simulink model "Mission_Server_Swarm_2QDrone"  (Simulink 9.1)
settings: Solver=ode2  StartTime=0.0  StopTime=inf  FixedStep=0.001  RelTol=1e-3  EnableMultiTasking=on
undefined symbols (not defined in the file): Host, qc_get_step_size
libraries: quarc_library x31, simulink x8
(part 2 of 2)

== system Mission_Server_Swarm_2QDrone/MISSION SERVER QDRONE SWARM/Communications Check/Triggered Subsystem1 ==
  note: This looks for the first falling edge to trigger a communication issue,
      | because the mission server model starts first.
  Trigger : TriggerPort  TriggerType=falling  VariantControl=Variant
  Add : Sum
  Compare To Constant : simulink/Logic and Bit Operations/Compare To Constant  relop=>=  const=1  OutDataTypeStr=boolean
  Constant : Constant
  Memory : Memory  InheritSampleTime=on
  Communication Issue (0,1) : Outport  InitialOutput=0
  wires:
  Compare To Constant/1 -> Communication Issue (0,1)/1
  Add/1 -> Memory/1, Compare To Constant/1
  Memory/1 -> Add/2
  Constant/1 -> Add/1

== system Mission_Server_Swarm_2QDrone/MISSION SERVER QDRONE SWARM/Data Server (Localization) /Convention Correction (Motive Frame to Research Studio Frame) - Drone 1 ==
  note: MF_R_RSF
  note: This subsystem converts measurements in the Motive Frame (MF)(raw optitrack) into the Research Studio Frame (RSF).
  note: RSF_R_MF
  note: XYZ in MF
  note: RPY in MF
  note: position
  note: attitude
  note: XYZ in RSF
  note: RPY in RSF
  xyz_MF (m) [3] : Inport
  rot_MF (rad) [3] : Inport  Port=2
  Inverse of  Orthonormal  Matrix is its  Transpose : Math  Operator=transpose  SaturateOnIntegerOverflow=on
  Prevent Gimbal Lock : Subsystem
  Product : Product  Multiplication=Matrix(*)
  Product1 : Product  Multiplication=Matrix(*)
  Rotate Basis from  RSF to MF : Constant  Value=[0 -1 0;0 0 1;-1 0 0]
  xyz_RSF (m) [3] : Outport
  rot_RSF (rad) [3] : Outport  Port=2
  wires:
  Rotate Basis from  RSF to MF/1 -> Inverse of  Orthonormal  Matrix is its  Transpose/1
  xyz_MF (m) [3]/1 -> Product1/2
  Inverse of  Orthonormal  Matrix is its  Transpose/1 -> Product1/1, Product/1
  rot_MF (rad) [3]/1 -> Product/2
  Product1/1 -> xyz_RSF (m) [3]/1
  Product/1 -> Prevent Gimbal Lock/1(Attitude (rad) [3])
  Prevent Gimbal Lock/1("Attitude (rad) [3] ") -> rot_RSF (rad) [3]/1

== system Mission_Server_Swarm_2QDrone/MISSION SERVER QDRONE SWARM/Data Server (Localization) /Convention Correction (Motive Frame to Research Studio Frame) - Drone 2 ==
  note: RPY in RSF
  note: XYZ in RSF
  note: attitude
  note: position
  note: RPY in MF
  note: XYZ in MF
  note: RSF_R_MF
  note: This subsystem converts measurements in the Motive Frame (MF)(raw optitrack) into the Research Studio Frame (RSF).
  note: MF_R_RSF
  xyz_MF (m) [3] : Inport
  rot_MF (rad) [3] : Inport  Port=2
  Inverse of  Orthonormal  Matrix is its  Transpose : Math  Operator=transpose  SaturateOnIntegerOverflow=on
  Prevent Gimbal Lock : Subsystem
  Product : Product  Multiplication=Matrix(*)
  Product1 : Product  Multiplication=Matrix(*)
  Rotate Basis from  RSF to MF : Constant  Value=[0 -1 0;0 0 1;-1 0 0]
  xyz_RSF (m) [3] : Outport
  rot_RSF (rad) [3] : Outport  Port=2
  wires:
  Prevent Gimbal Lock/1("Attitude (rad) [3] ") -> rot_RSF (rad) [3]/1
  Product/1 -> Prevent Gimbal Lock/1(Attitude (rad) [3])
  Product1/1 -> xyz_RSF (m) [3]/1
  rot_MF (rad) [3]/1 -> Product/2
  Inverse of  Orthonormal  Matrix is its  Transpose/1 -> Product/1, Product1/1
  xyz_MF (m) [3]/1 -> Product1/2
  Rotate Basis from  RSF to MF/1 -> Inverse of  Orthonormal  Matrix is its  Transpose/1

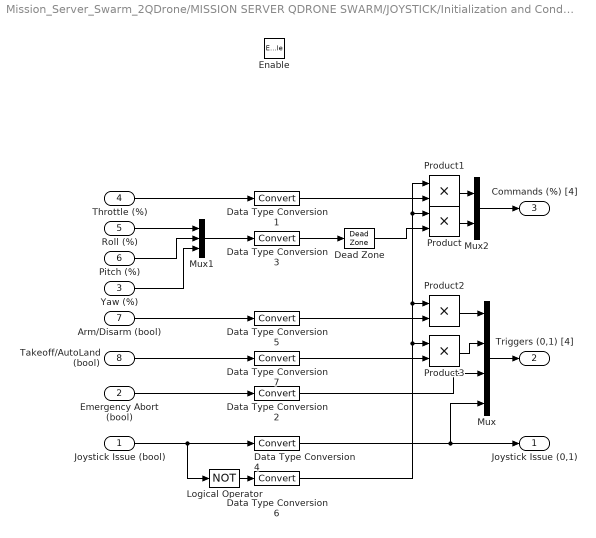
== system Mission_Server_Swarm_2QDrone/MISSION SERVER QDRONE SWARM/JOYSTICK/Initialization and Conditioning ==
  Joystick Issue (bool) : Inport
  Emergency Abort (bool) : Inport  Port=2
  Yaw (%) : Inport  Port=3
  Throttle (%) : Inport  Port=4
  Roll (%) : Inport  Port=5
  Pitch (%) : Inport  Port=6
  Arm/Disarm (bool) : Inport  Port=7
  Takeoff/AutoLand (bool) : Inport  Port=8
  Enable : EnablePort  StatesWhenEnabling=reset
  Data Type Conversion{1..7} (7 alike) : DataTypeConversion
  Dead Zone : DeadZone  LowerValue=-0.01  UpperValue=0.01  SaturateOnIntegerOverflow=on
  Logical Operator : Logic  Operator=NOT  AllPortsSameDT=off  OutDataTypeStr=boolean
  Mux : Mux
  Mux1 : Mux  Inputs=3
  Mux2 : Mux  Inputs=2
  Product{,1..3} (4 alike) : Product
  Joystick Issue (0,1) : Outport  InitialOutput=0
  Triggers (0,1) [4] : Outport  Port=2  InitialOutput=0
  Commands (%) [4] : Outport  Port=3  InitialOutput=0
  wires:
  Mux2/1 -> Commands (%) [4]/1
  Data Type Conversion7/1 -> Product3/2
  Product3/1 -> Mux/2
  Takeoff/AutoLand (bool)/1 -> Data Type Conversion7/1
  Data Type Conversion5/1 -> Product2/2
  Product2/1 -> Mux/1
  Data Type Conversion6/1 -> Product3/1, Product2/1, Product/1, Product1/1
  Dead Zone/1 -> Product/2
  Data Type Conversion1/1 -> Product1/2
  Product1/1 -> Mux2/1
  Product/1 -> Mux2/2
  Logical Operator/1 -> Data Type Conversion6/1
  Data Type Conversion2/1 -> Mux/3
  Mux/1 -> Triggers (0,1) [4]/1
  Arm/Disarm (bool)/1 -> Data Type Conversion5/1
  Data Type Conversion3/1 -> Dead Zone/1
  Emergency Abort (bool)/1 -> Data Type Conversion2/1
  Data Type Conversion4/1 -> Joystick Issue (0,1)/1, Mux/4
  Yaw (%)/1 -> Mux1/3
  Pitch (%)/1 -> Mux1/2
  Roll (%)/1 -> Mux1/1
  Throttle (%)/1 -> Data Type Conversion1/1
  Mux1/1 -> Data Type Conversion3/1
  Joystick Issue (bool)/1 -> Logical Operator/1, Data Type Conversion4/1

== system Mission_Server_Swarm_2QDrone/MISSION SERVER QDRONE SWARM/JOYSTICK/Pulse Check ==
  note: For this subsystem we will count the number of new pulses. The data can be considered enabled once the count of new signals has gone beyond 2. This will enable the Initializing and conditioning subsystem.
  new : Inport
  Compare : quarc_library/Logic Operations/Compare  operator=>  output_data_type=boolean
      settings: SourceProductName=QUARC Targets
  Pulse Check : Constant  Value=2
  "pulse count " : Subsystem  TreatAsAtomicUnit=on
  signal enable : Outport  InitialOutput=0
  wires:
  Compare/1 -> signal enable/1
  Pulse Check/1 -> Compare/2
  new/1 -> "pulse count "/Trigger
  "pulse count "/1(Number of Pulses) -> Compare/1

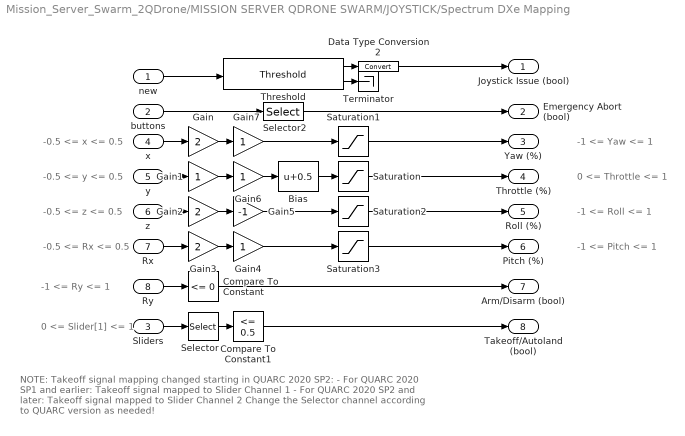
== system Mission_Server_Swarm_2QDrone/MISSION SERVER QDRONE SWARM/JOYSTICK/Spectrum DXe Mapping ==
  note: NOTE: Takeoff signal mapping changed starting in QUARC 2020 SP2:
      |
      | - For QUARC 2020 SP1 and earlier: Takeoff signal mapped to Slider Channel 1
      | - For QUARC 2020 SP2 and later: Takeoff signal mapped to Slider Channel 2
      |
      | Change the Selector channel according to QUARC version as needed!
  note: -1 <= Ry <= 1
  note: 0 <= Slider[1] <= 1
  note: -1 <= Pitch <= 1
  note: -0.5 <= Rx <= 0.5
  note: -1 <= Roll <= 1
  note: -0.5 <= z <= 0.5
  note: 0 <= Throttle <= 1
  note: -0.5 <= y <= 0.5
  note: -1 <= Yaw <= 1
  note: -0.5 <= x <= 0.5
  new : Inport
  buttons : Inport  Port=2
  Sliders : Inport  Port=3
  x : Inport  Port=4
  y : Inport  Port=5
  z : Inport  Port=6
  Rx : Inport  Port=7
  Ry : Inport  Port=8
  Bias : Bias  Bias=0.5
  Compare To Constant : simulink/Logic and Bit Operations/Compare To Constant  relop=<=  const=0  OutDataTypeStr=boolean
  Compare To Constant1 : simulink/Logic and Bit Operations/Compare To Constant  relop=<=  const=0.5  OutDataTypeStr=boolean
  Data Type Conversion2 : DataTypeConversion
  Gain : Gain  Gain=2
  Gain{1,4,6..7} (4 alike) : Gain
  Gain2 : Gain  Gain=2
  Gain3 : Gain  Gain=2
  Gain5 : Gain  Gain=-1
  Saturation : Saturate  UpperLimit=1  LowerLimit=0
  Saturation1 : Saturate  UpperLimit=1  LowerLimit=-1
  Saturation2 : Saturate  UpperLimit=1  LowerLimit=-1
  Saturation3 : Saturate  UpperLimit=1  LowerLimit=-1
  Selector : Selector  InputPortWidth=2  IndexOptions=Index vector (dialog)  Indices=[2]  OutputSizes=1
  Selector2 : Selector  InputPortWidth=32  IndexOptions=Index vector (dialog)  Indices=[1]  OutputSizes=1
  Terminator : Terminator
  Threshold : quarc_library/Discontinuities/Threshold  operator===  param_src=Specify via dialog  threshold=0  duration=1
      settings: SourceProductName=QUARC Targets
  Joystick Issue (bool) : Outport
  Emergency Abort (bool) : Outport  Port=2
  Yaw (%) : Outport  Port=3
  Throttle (%) : Outport  Port=4
  Roll (%) : Outport  Port=5
  Pitch (%) : Outport  Port=6
  "Arm/Disarm (bool) " : Outport  Port=7
  Takeoff/Autoland (bool) : Outport  Port=8
  wires:
  Data Type Conversion2/1 -> Joystick Issue (bool)/1
  new/1 -> Threshold/1
  Threshold/1 -> Data Type Conversion2/1
  Selector2/1 -> Emergency Abort (bool)/1
  Threshold/2 -> Terminator/1
  buttons/1 -> Selector2/1
  Compare To Constant1/1 -> Takeoff/Autoland (bool)/1
  Rx/1 -> Gain3/1
  y/1 -> Gain1/1
  Ry/1 -> Compare To Constant/1
  x/1 -> Gain/1
  z/1 -> Gain2/1
  Gain4/1 -> Saturation3/1
  Gain1/1 -> Gain6/1
  Gain2/1 -> Gain5/1
  Bias/1 -> Saturation/1
  Saturation2/1 -> Roll (%)/1
  Gain3/1 -> Gain4/1
  Gain/1 -> Gain7/1
  Saturation1/1 -> Yaw (%)/1
  Gain6/1 -> Bias/1
  Sliders/1 -> Selector/1
  Saturation/1 -> Throttle (%)/1
  Gain5/1 -> Saturation2/1
  Selector/1 -> Compare To Constant1/1
  Gain7/1 -> Saturation1/1
  Saturation3/1 -> Pitch (%)/1
  Compare To Constant/1 -> "Arm/Disarm (bool) "/1

== system Mission_Server_Swarm_2QDrone/MISSION SERVER QDRONE SWARM/Data Server (Localization) /Convention Correction (Motive Frame to Research Studio Frame) - Drone 1/Prevent Gimbal Lock ==
  note: Remapping the rotation order to prevent gimbal lock
      | in heading/yaw due to Euler singularity condition
  Attitude (rad) [3] : Inport
  Demux : Demux  Outputs=3
  Euler Angles from Rotation Matrix (Relative ZYX) : quarc_library/Math Operations/Matrices/Euler Angles from Rotation Matrix  menu_order=Relative Z-Y-X
      settings: SourceProductName=QUARC Targets
  Euler Angles to Rotation Matrix (Relative YZX) : quarc_library/Math Operations/Matrices/Euler Angles to Rotation Matrix  menu_order=Relative Y-Z-X
      settings: SourceProductName=QUARC Targets
  Mux : Mux  Inputs=3
  "Attitude (rad) [3] " : Outport
  wires:
  Euler Angles from Rotation Matrix (Relative ZYX)/2 -> Mux/2
  Euler Angles from Rotation Matrix (Relative ZYX)/1 -> Mux/3
  Euler Angles from Rotation Matrix (Relative ZYX)/3 -> Mux/1
  Euler Angles to Rotation Matrix (Relative YZX)/1 -> Euler Angles from Rotation Matrix (Relative ZYX)/1
  Attitude (rad) [3]/1 -> Demux/1
  Mux/1 -> "Attitude (rad) [3] "/1
  Demux/2 -> Euler Angles to Rotation Matrix (Relative YZX)/1
  Demux/3 -> Euler Angles to Rotation Matrix (Relative YZX)/2
  Demux/1 -> Euler Angles to Rotation Matrix (Relative YZX)/3

== system Mission_Server_Swarm_2QDrone/MISSION SERVER QDRONE SWARM/Data Server (Localization) /Convention Correction (Motive Frame to Research Studio Frame) - Drone 2/Prevent Gimbal Lock ==
  note: Remapping the rotation order to prevent gimbal lock
      | in heading/yaw due to Euler singularity condition
  Attitude (rad) [3] : Inport
  Demux : Demux  Outputs=3
  Euler Angles from Rotation Matrix (Relative ZYX) : quarc_library/Math Operations/Matrices/Euler Angles from Rotation Matrix  menu_order=Relative Z-Y-X
      settings: SourceProductName=QUARC Targets
  Euler Angles to Rotation Matrix (Relative YZX) : quarc_library/Math Operations/Matrices/Euler Angles to Rotation Matrix  menu_order=Relative Y-Z-X
      settings: SourceProductName=QUARC Targets
  Mux : Mux  Inputs=3
  "Attitude (rad) [3] " : Outport
  wires:
  Demux/1 -> Euler Angles to Rotation Matrix (Relative YZX)/3
  Demux/3 -> Euler Angles to Rotation Matrix (Relative YZX)/2
  Demux/2 -> Euler Angles to Rotation Matrix (Relative YZX)/1
  Mux/1 -> "Attitude (rad) [3] "/1
  Attitude (rad) [3]/1 -> Demux/1
  Euler Angles to Rotation Matrix (Relative YZX)/1 -> Euler Angles from Rotation Matrix (Relative ZYX)/1
  Euler Angles from Rotation Matrix (Relative ZYX)/3 -> Mux/1
  Euler Angles from Rotation Matrix (Relative ZYX)/1 -> Mux/3
  Euler Angles from Rotation Matrix (Relative ZYX)/2 -> Mux/2

== system Mission_Server_Swarm_2QDrone/MISSION SERVER QDRONE SWARM/JOYSTICK/Pulse Check/pulse count  ==
  Trigger : TriggerPort  VariantControl=Variant
  Constant1 : Constant  Value=0
  Increment Stored Integer : simulink/Additional Math & Discrete/Additional Math: Increment - Decrement/Increment Stored Integer
  Sum : Sum  Inputs=|++
  Unit Delay : UnitDelay  SampleTime=-1
  Number of Pulses : Outport
  wires:
  Constant1/1 -> Sum/1
  Sum/1 -> Increment Stored Integer/1
  Unit Delay/1 -> Sum/2
  Increment Stored Integer/1 -> Unit Delay/1, Number of Pulses/1

== matlab function MISSION SERVER QDRONE SWARM/n vehicles Circular Trajectories/generate vector of 0s for Yaw ==
  data: u input double; y output double
function y = fcn(u)

y = 0.*u;

== matlab function MISSION SERVER QDRONE SWARM/n vehicles Circular Trajectories/generate vector of 1s ==
  data: u input double; y output double
function y = fcn(u)

y = 0.*u + 1;

== matlab function MISSION SERVER QDRONE SWARM/n vehicles Circular Trajectories/variable size reshape ==
  data: u input double; y output double
function y = fcn(u)
y = u;
num = length(u)/4;
for i = 1:4
    for j = 1:num
        y(4*(j-1) + i) = u(j + num*(i-1));
    end
end

== matlab function Communication V1/Detect Communication loss/MATLAB Function ==
  data: time input double; stream_connection_loss output double; state input double; error input double
function stream_connection_loss  = fcn(time, state, error)

stream_connection_loss = 0;
if time > 1
    if ~((state == 2)&&(error >= 0))
        % stream connection is not established correctly
        stream_connection_loss = 1;
    end
end

== matlab function Communication V2/Detect Communication loss/MATLAB Function ==
  data: time input double; stream_connection_loss output double; state input double; error input double
function stream_connection_loss  = fcn(time, state, error)

stream_connection_loss = 0;
if time > 1
    if ~((state == 2)&&(error >= 0))
        % stream connection is not established correctly
        stream_connection_loss = 1;
    end
end

== matlab function MISSION SERVER QDRONE SWARM/Extract Vehicle Data 7/Extract Object Data ==
  data: data input double; position output double; orientation output double; index input double; tracking output double
function [position, orientation, tracking] = fcn(data, index)

n = length(data)/7;

if (index<=0)||(index>n)
    position = zeros(1,3); orientation = zeros(1,3); tracking = 0;
else
    position = [data(index*3-2), data(index*3-1), data(index*3)];
    orientation = [data((index+n)*3 - 2), data((index+n)*3 - 1), data((index+n)*3)];
    tracking = data(index + (n*6));
end

== matlab function MISSION SERVER QDRONE SWARM/Extract Vehicle Data 1/Extract Object Data ==
  data: data input double; position output double; orientation output double; index input double; tracking output double
function [position, orientation, tracking] = fcn(data, index)

n = length(data)/7;

if (index<=0)||(index>n)
    position = zeros(1,3); orientation = zeros(1,3); tracking = 0;
else
    position = [data(index*3-2), data(index*3-1), data(index*3)];
    orientation = [data((index+n)*3 - 2), data((index+n)*3 - 1), data((index+n)*3)];
    tracking = data(index + (n*6));
end

== matlab function MISSION SERVER QDRONE SWARM/Extract Vehicle Data 2/Extract Object Data ==
  data: data input double; position output double; orientation output double; index input double; tracking output double
function [position, orientation, tracking] = fcn(data, index)

n = length(data)/7;

if (index<=0)||(index>n)
    position = zeros(1,3); orientation = zeros(1,3); tracking = 0;
else
    position = [data(index*3-2), data(index*3-1), data(index*3)];
    orientation = [data((index+n)*3 - 2), data((index+n)*3 - 1), data((index+n)*3)];
    tracking = data(index + (n*6));
end
